simulink model "arduino_interfacing"  (R2026a)
settings: Solver=FixedStepAuto  StopTime=50.0  EnableMultiTasking=on
libraries: arduinolib x2
settings Model: SimulationMode=external  SILPILModeSetting=veronly  ExtModeTrigDuration=2  Creator=ejarr  LastModifiedBy=ejarr
settings HardwareCC: ProdBitPerInt=16.0  ProdBitPerPointer=16.0  ProdBitPerSizeT=16.0  ProdBitPerPtrDiffT=16.0  ProdWordSize=8.0  ProdHWDeviceType=Atmel->AVR  UseEmbeddedCoderFeatures=off  UseSimulinkCoderFeatures=off
settings RTWCC: SystemTargetFile=ert.tlc  HardwareBoard=Arduino Mega 2560  TLCOptions=-aInlineSetEventsForThisBaseRateFcn=TLC_FALSE -aSuppressMultiTaskScheduler=TLC_FALSE -aRateBasedStepFcn=1  Toolchain=Arduino AVR  BuildConfiguration=Faster Runs  Description=Embedded Coder
settings CodeAppCC: MangleLength=10.0
settings ERTTargetCC: ExtModeTransport=3.0  ExtModeAutomaticAllocSize=off  ExtModeStaticAllocSize=2048.0  SupportContinuousTime=on  SupportNonInlinedSFcns=on  SupportVariableSizeSignals=on

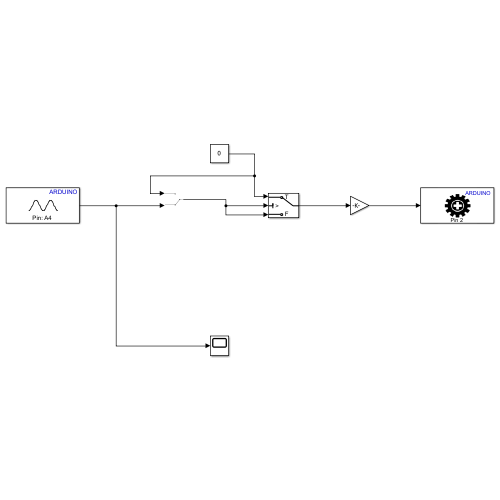
[thumbnail: Simulink's stored preview of the top-level diagram]
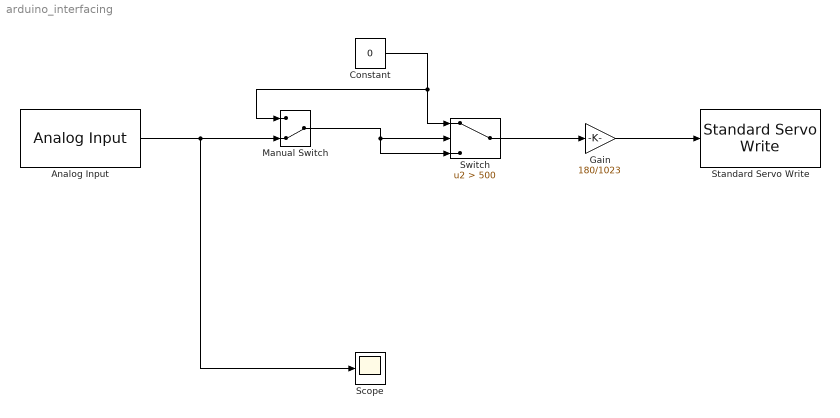
== system arduino_interfacing ==
  Analog Input : arduinolib/Analog Input  pinNumber=4  ReadResultsOnly=off  ConversionTriggerSource=Software  ExternalTriggerType=uint32( 0 )  OutputDataType=uint16  EnableConversionCompleteNotify=off  EnableOuputStatus=off  SampleTime=-1  blockPlatform=arduino
      settings: LibrarySourceBlock=gizmoLibrary/Arduino Utilities/Analog Input
  Constant : Constant  Value=0
  Gain : Gain  Gain=180/1023  OutDataTypeStr=double
  Manual Switch : ManualSwitch  CurrentSetting=0
  Scope : Scope
      settings: ActiveDisplayYMinimum=-10.249999999999986  ActiveDisplayYMaximum=762.25
  Standard Servo Write : arduinolib/Standard Servo Write  pinNumber=2  ServoIndex=0  blockPlatform=ARDUINO
  Switch : Switch  Criteria=u2 > Threshold  Threshold=500  SaturateOnIntegerOverflow=off  InputSameDT=off
  wires:
  Gain/1 -> Standard Servo Write/1
  Switch/1 -> Gain/1
  Constant/1 -> Manual Switch/1, Switch/1
  Analog Input/1 -> Manual Switch/2, Scope/1
  Manual Switch/1 -> Switch/2, Switch/3
